simulink model "EV6_LUT_FourWheel_EV6Battery77p4kWh_PowerCorrected"  (R2024a)
settings: Solver=ode4  StartTime=0  StopTime=60  FixedStep=0.001  RelTol=1e-3
PreLoadFcn:
  | VSS_BICYCLE=Simulink.Variant('Dual=0');
  | VSS_DUAL=Simulink.Variant('Dual=1');
  | Dual=1;
  | load('DriveCycle2.mat')
PostLoadFcn:
  | if any(exist('dsrtsu_mdlpostloadfcn', 'file') ~= 0), dsrtsu_mdlpostloadfcn('Execute', bdroot); end
InitFcn:
  | , if any(exist('rtifpga_mdlclblib', 'file') ~= 0), rtifpga_mdlclblib('Init', bdroot); end,
  | , if any(exist('dsmpb_private', 'file') ~= 0), dsmpb_private('dsmpb_mdlclblib', 'Init', bdroot); end,
  | load('DriveCycle2.mat')
model workspace (MAT data in the model file):
  DiffRatio = 10.65
  EV6_2023_BattBranchCapacity_Ah = 55.5236728838
  EV6_2023_BattEnergy_kWh = 77.4
  EV6_2023_BattNominalVoltage_V = 697
  EV6_2023_BattNumCellsParallel = 2
  EV6_2023_BattNumCellsSeries = 192
  EV6_2023_BattOpenVoltCapBpts = [0 0.1 0.2 0.3 0.4 0.5 0.6 0.7 0.8 0.9 1]
  EV6_2023_BattOpenVoltTbl = [2.96762142548 3.40364281191 3.47417488548 3.54470541822 3.61523441014 3.68576186124 3.75628777151 3.82681214095 3.94527005036 4.07101207308 4.2120755254]
  EV6_2023_BattPackCapacity_Ah = 111.047345768
  EV6_2023_BattResistSocBpts = [0 0.2 0.4 0.6 0.8 1]
  EV6_2023_BattResistTbl = [0.0163620057716 0.0118174152018 0.00807187352333 0.00375663957972 0.00266904525531 0.00103635901355 0.0019014404175 0.0172368903217 0.0121226074867 0.00758541551769 0.00474065349228 0.00337561163613 ... (42 elements, 7x6)]
  EV6_2023_BattResistTempBpts = [243.1 253.1 263.1 273.1 283.1 298.1 313.1]
  EV6_2023_InitialPackOCV_V = 726.471714233
  EV6_2023_InitialSOC = 0.638878863672
  EV6_BattCellCapacity_Ah = 60.3
  EV6_BattInitialSOC = 0.638878863672
  EV6_BattOCV_Cell_V = [2.96762142548 3.40364281191 3.47417488548 3.54470541822 3.61523441014 3.68576186124 3.75628777151 3.82681214095 3.94527005036 4.07101207308 4.2120755254]
  EV6_BattOCV_SOC = [0 0.1 0.2 0.3 0.4 0.5 0.6 0.7 0.8 0.9 1]
  EV6_BattPackCapacity_Ah = 120.6
  EV6_BattParallelCells = 2
  EV6_BattResistanceSOC = [0 0.2 0.4 0.6 0.8 1]
  EV6_BattResistanceTable_Ohm = [0.0163620057716 0.0118174152018 0.00807187352333 0.00375663957972 0.00266904525531 0.00103635901355 0.0019014404175 0.0172368903217 0.0121226074867 0.00758541551769 0.00474065349228 0.00337561163613 ... (42 elements, 7x6)]
  EV6_BattResistanceTemp_K = [243.1 253.1 263.1 273.1 283.1 298.1 313.1]
  EV6_BattSeriesCells = 192
  EV6_FinalDriveRatio = 10.65
  EV6_TargetPackResistance_Ohm = 0.132763804608
  Gas = 0.383333333333
undefined symbols (not defined in the file): accel_bp_mps2, AccelCmd, ActTqLF_Nm_, ActTqLR_Nm_, ActTqRF_Nm_, ActTqRR_Nm_, BattChargeLimitMaxPwr, BattChargeLimitSocBpts, BattChargeLimitTbl, BattDischargeLimitSocBpts, BattDischargeLimitTbl, BattDischargeMaxPwr, BrakeMaxPrs, BrakeMaxTrq, ChassisDistCg2FrontAxle, ChassisDistCg2RearAxle, ChassisVehMass, CltchCmd, CoastDown, DecelCmd, DiscIntNeverNeededParam, EnvGravCnst, EnvPrs, EnvTemp, EV6_RegenTorqueGain, EV6_TractionTorqueGain, front_share_regen_3d, front_share_traction_3d, FuelSpecificGrav, GearCmd, h, InitStates, lgSw, limitedMCT, MCT, MtrEffSpdBpts, MtrEffTbl, MtrEffTrqBpts, MtrPwrMax, MtrTrqMax, out_1, pMCT, RealSimPara, Ref_speed, Ref_time, regen_torque_bp_Nm, speed_bp_kph, SteeringCmd, SupvsryCtrlRegenBrkCutOffTbl, SupvsryCtrlRegenSpdBpts, TestScnrioCycleNum, traction_torque_bp_Nm, US06, VEH
libraries: VSIGenLib x65, simulink x54, etargetslib x38, dsmpblib x24, vehdynlibtire x12, autolibshared x11, vehdynlibsuspension x7, vehdynlibtirecommon x7, autolibpowerinfoutils x6, autolibutils x5, autolibsharedcoupling x4, autolibmappedmotor x4
(part 18 of 19)

== system EV6_LUT_FourWheel_EV6Battery77p4kWh_PowerCorrected/Vehicle Under Test1/Vehicle/Vehicle Dynamics/Vehicle 14DOF/Wheels and Tires/VDBS/Veh2Tire/Wheel Angles ==
  steer : Inport
  camber : Inport  Port=2
  Add1 : Sum
  Add2 : Sum
  Constant1 : Constant  Value=pi
  Constant2 : Constant  Value=[pi;0;pi;0].*0+[0;pi;0;pi].*0
  Constant3 : Constant  Value=ones(1,4).*0
  Reshape : Reshape  OutputDimensionality=Row vector (2-D)
  Reshape1 : Reshape  OutputDimensionality=Row vector (2-D)
  Reshape2 : Reshape  OutputDimensionality=Row vector (2-D)
  Vector Concatenate3 : Concatenate  NumInputs=3  Mode=Multidimensional array
  Vehicle : Outport  VectorParamsAs1DForOutWhenUnconnected=off
  wires:
  Add2/1 -> Reshape1/1
  Constant1/1 -> Add2/2
  Add1/1 -> Reshape/1
  steer/1 -> Add1/1
  Reshape2/1 -> Vector Concatenate3/2
  camber/1 -> Add2/1
  Reshape1/1 -> Vector Concatenate3/1
  Reshape/1 -> Vector Concatenate3/3
  Vector Concatenate3/1 -> Vehicle/1
  Constant3/1 -> Reshape2/1
  Constant2/1 -> Add1/2

== system EV6_LUT_FourWheel_EV6Battery77p4kWh_PowerCorrected/Vehicle Under Test1/Vehicle/Vehicle Dynamics/Vehicle 14DOF/Wheels and Tires/VDBS/Veh2Tire/Wheel to Body Transform ==
  VelVeh : Inport  Partition=on  PartitionDimension=2  PartitionWidth=1  PartitionOffset=0
  WheelAngles : Inport  Port=2  Partition=on  PartitionDimension=2  PartitionWidth=1  PartitionOffset=0
  Demux1 : Demux  Outputs=3
  Divide1 : Product  Inputs=**  Multiplication=Matrix(*)
  For Each : ForEach  DisableCoverage=on
  Rotation Angles to Direction Cosine Matrix Retro: ZYX : Subsystem
  Selector : Selector  InputPortWidth=3  IndexOptions=Index vector (dialog)  Indices=[3 2 1]  OutputSizes=1
  xdotWheel : Outport  ConcatenationDimension=1  VectorParamsAs1DForOutWhenUnconnected=off
  ydotWheel : Outport  Port=2  ConcatenationDimension=1  VectorParamsAs1DForOutWhenUnconnected=off
  zdotWheel : Outport  Port=3  ConcatenationDimension=1  VectorParamsAs1DForOutWhenUnconnected=off
  wires:
  Selector/1 -> Rotation Angles to Direction Cosine Matrix Retro: ZYX/1(In1)
  WheelAngles/1 -> Selector/1
  VelVeh/1 -> Divide1/2
  Rotation Angles to Direction Cosine Matrix Retro: ZYX/1(Out1) -> Divide1/1
  Demux1/3 -> zdotWheel/1
  Demux1/2 -> ydotWheel/1
  Demux1/1 -> xdotWheel/1
  Divide1/1 -> Demux1/1

== system EV6_LUT_FourWheel_EV6Battery77p4kWh_PowerCorrected/Vehicle Under Test1/Vehicle/Vehicle Dynamics/Vehicle 7DOF/Longitudinal Wheels 4DOF/Velocity and Vertical Load/Bicycle/Bicycle Fz ==
  In1 : Inport
  Bus Selector6 : BusSelector  OutputSignals=BdyFrm.Forces.Tires.FrntTire.Fz,BdyFrm.Forces.Tires.RearTire.Fz
  Cont LPF : autolibutils/Cont LPF  wc=20*2*pi  AbsoluteTolerance=auto  aMode=2
  Mux5 : Mux
  Saturation : Saturate  UpperLimit=20e3  LowerLimit=1000  ZeroCross=off
  Out1 : Outport  VectorParamsAs1DForOutWhenUnconnected=off
  wires:
  Mux5/1 -> Saturation/1
  Bus Selector6/1 -> Mux5/1, Mux5/2  "<Fz>"
  In1/1 -> Bus Selector6/1
  Bus Selector6/2 -> Mux5/3, Mux5/4  "<Fz>"
  Saturation/1 -> Cont LPF/1
  Cont LPF/1 -> Out1/1

== system EV6_LUT_FourWheel_EV6Battery77p4kWh_PowerCorrected/Vehicle Under Test1/Vehicle/Vehicle Dynamics/Vehicle 7DOF/Longitudinal Wheels 4DOF/Velocity and Vertical Load/Bicycle/Bicycle V ==
  In1 : Inport
  Bus Selector : BusSelector  OutputSignals=BdyFrm.FrntAxl.Vel.xdot,BdyFrm.FrntAxl.Vel.ydot,BdyFrm.FrntAxl.Vel.zdot  OutputAsBus=on
  Bus Selector3 : BusSelector  OutputSignals=BdyFrm.RearAxl.Vel.xdot,BdyFrm.RearAxl.Vel.ydot,BdyFrm.RearAxl.Vel.zdot  OutputAsBus=on
  Bus to Vector1 : BusToVector
  Bus to Vector3 : BusToVector
  Vector Concatenate1 : Concatenate  NumInputs=4  Mode=Multidimensional array  ConcatenateDimension=2
  Out1 : Outport  VectorParamsAs1DForOutWhenUnconnected=off
  wires:
  Vector Concatenate1/1 -> Out1/1
  Bus to Vector3/1 -> Vector Concatenate1/3, Vector Concatenate1/4
  Bus Selector/1 -> Bus to Vector1/1
  In1/1 -> Bus Selector/1, Bus Selector3/1
  Bus to Vector1/1 -> Vector Concatenate1/1, Vector Concatenate1/2
  Bus Selector3/1 -> Bus to Vector3/1

== system EV6_LUT_FourWheel_EV6Battery77p4kWh_PowerCorrected/Vehicle Under Test1/Vehicle/Vehicle Dynamics/Vehicle 7DOF/Longitudinal Wheels 4DOF/Velocity and Vertical Load/Dual/Dual Fz ==
  In1 : Inport
  Bus Selector6 : BusSelector  OutputSignals=BdyFrm.Forces.Tires.FrntTires.Lft.Fz,BdyFrm.Forces.Tires.FrntTires.Rght.Fz,BdyFrm.Forces.Tires.RearTires.Lft.Fz,BdyFrm.Forces.Tires.RearTires.Rght.Fz
  Cont LPF : autolibutils/Cont LPF  wc=20*2*pi  AbsoluteTolerance=auto  aMode=2
  Saturation : Saturate  UpperLimit=20e3  LowerLimit=1000  ZeroCross=off
  Vector Concatenate : Concatenate  NumInputs=4
  Out1 : Outport  VectorParamsAs1DForOutWhenUnconnected=off
  wires:
  Bus Selector6/4 -> Vector Concatenate/4  "<Fz>"
  Bus Selector6/3 -> Vector Concatenate/3  "<Fz>"
  Bus Selector6/1 -> Vector Concatenate/1  "<Fz>"
  Bus Selector6/2 -> Vector Concatenate/2  "<Fz>"
  Vector Concatenate/1 -> Saturation/1
  Cont LPF/1 -> Out1/1
  Saturation/1 -> Cont LPF/1
  In1/1 -> Bus Selector6/1

== system EV6_LUT_FourWheel_EV6Battery77p4kWh_PowerCorrected/Vehicle Under Test1/Vehicle/Vehicle Dynamics/Vehicle 7DOF/Longitudinal Wheels 4DOF/Velocity and Vertical Load/Dual/Dual V ==
  In1 : Inport
  Bus Selector1 : BusSelector  OutputSignals=BdyFrm.FrntAxl.Lft.Vel.xdot,BdyFrm.FrntAxl.Lft.Vel.ydot,BdyFrm.FrntAxl.Lft.Vel.zdot  OutputAsBus=on
  Bus Selector2 : BusSelector  OutputSignals=BdyFrm.FrntAxl.Rght.Vel.xdot,BdyFrm.FrntAxl.Rght.Vel.ydot,BdyFrm.FrntAxl.Rght.Vel.zdot  OutputAsBus=on
  Bus Selector4 : BusSelector  OutputSignals=BdyFrm.RearAxl.Lft.Vel.xdot,BdyFrm.RearAxl.Lft.Vel.ydot,BdyFrm.RearAxl.Lft.Vel.zdot  OutputAsBus=on
  Bus Selector5 : BusSelector  OutputSignals=BdyFrm.RearAxl.Rght.Vel.xdot,BdyFrm.RearAxl.Rght.Vel.ydot,BdyFrm.RearAxl.Rght.Vel.zdot  OutputAsBus=on
  Bus to Vector{5..8} (4 alike) : BusToVector
  Vector Concatenate2 : Concatenate  NumInputs=4  Mode=Multidimensional array  ConcatenateDimension=2
  Out1 : Outport  VectorParamsAs1DForOutWhenUnconnected=off
  wires:
  Vector Concatenate2/1 -> Out1/1
  Bus to Vector7/1 -> Vector Concatenate2/3
  Bus Selector5/1 -> Bus to Vector8/1
  In1/1 -> Bus Selector5/1, Bus Selector4/1, Bus Selector2/1, Bus Selector1/1
  Bus Selector1/1 -> Bus to Vector5/1
  Bus to Vector5/1 -> Vector Concatenate2/1
  Bus Selector4/1 -> Bus to Vector7/1
  Bus to Vector8/1 -> Vector Concatenate2/4
  Bus Selector2/1 -> Bus to Vector6/1
  Bus to Vector6/1 -> Vector Concatenate2/2

== system EV6_LUT_FourWheel_EV6Battery77p4kWh_PowerCorrected/Vehicle Under Test1/Vehicle/Vehicle Dynamics/Vehicle 14DOF/Wheels and Tires/VDBS/Tire2Veh/Wheel to Body Transform/Rotation Angles to Direction Cosine Matrix Retro: ZYX ==
  In1 : Inport
  Fcn : Fcn  Expr=u(5)*u(4)
  Fcn1 : Fcn  Expr=u(5)*u(1)
  Fcn2 : Fcn  Expr=-u(2)
  Fcn3 : Fcn  Expr=u(3)*u(2)*u(4)-u(6)*u(1)
  Fcn4 : Fcn  Expr=u(3)*u(2)*u(1)-u(6)*u(4)
  Fcn5 : Fcn  Expr=u(3)*u(5)
  Fcn6 : Fcn  Expr=u(6)*u(2)*u(4)-u(3)*u(1)
  Fcn7 : Fcn  Expr=u(6)*u(2)*u(1)-u(3)*u(4)
  Fcn8 : Fcn  Expr=u(6)*u(5)
  Mux : Mux  Inputs=2
  SinCos : Trigonometry  Operator=sincos
  Subsystem : Subsystem
  Out1 : Outport
  wires:
  Subsystem/1(Out1) -> Out1/1
  Fcn6/1 -> Subsystem/7(In7)
  Fcn3/1 -> Subsystem/4(In4)
  Fcn2/1 -> Subsystem/3(In3)
  Fcn5/1 -> Subsystem/6(In6)
  In1/1 -> SinCos/1
  Fcn4/1 -> Subsystem/5(In5)
  Fcn/1 -> Subsystem/1(In1)
  Fcn7/1 -> Subsystem/8(In8)
  Fcn8/1 -> Subsystem/9(In9)
  SinCos/1 -> Mux/1
  SinCos/2 -> Mux/2
  Mux/1 -> Fcn4/1, Fcn3/1, Fcn2/1, Fcn1/1, Fcn/1, Fcn5/1, Fcn6/1, Fcn7/1, Fcn8/1
  Fcn1/1 -> Subsystem/2(In2)

== system EV6_LUT_FourWheel_EV6Battery77p4kWh_PowerCorrected/Vehicle Under Test1/Vehicle/Vehicle Dynamics/Vehicle 14DOF/Wheels and Tires/VDBS/Tires/Fiala Tires/Fx ==
  In1 : Inport
  In2 : Inport  Port=2
  In3 : Inport  Port=3
  In4 : Inport  Port=4
  Bus Selector{,1..3} (4 alike) : BusSelector  OutputSignals=Fx
  Vector Concatenate : Concatenate  NumInputs=4
  Out1 : Outport  VectorParamsAs1DForOutWhenUnconnected=off
  wires:
  Vector Concatenate/1 -> Out1/1
  In1/1 -> Bus Selector/1
  Bus Selector/1 -> Vector Concatenate/1  "<Fx>"
  In2/1 -> Bus Selector1/1
  In3/1 -> Bus Selector2/1
  In4/1 -> Bus Selector3/1
  Bus Selector1/1 -> Vector Concatenate/2  "<Fx>"
  Bus Selector2/1 -> Vector Concatenate/3  "<Fx>"
  Bus Selector3/1 -> Vector Concatenate/4  "<Fx>"

== system EV6_LUT_FourWheel_EV6Battery77p4kWh_PowerCorrected/Vehicle Under Test1/Vehicle/Vehicle Dynamics/Vehicle 14DOF/Wheels and Tires/VDBS/Tires/Fiala Tires/Fy ==
  In1 : Inport
  In2 : Inport  Port=2
  In3 : Inport  Port=3
  In4 : Inport  Port=4
  Bus Selector{,1..3} (4 alike) : BusSelector  OutputSignals=Fy
  Vector Concatenate : Concatenate  NumInputs=4
  Out1 : Outport  VectorParamsAs1DForOutWhenUnconnected=off
  wires:
  Bus Selector3/1 -> Vector Concatenate/4  "<Fy>"
  Bus Selector2/1 -> Vector Concatenate/3  "<Fy>"
  Bus Selector1/1 -> Vector Concatenate/2  "<Fy>"
  In4/1 -> Bus Selector3/1
  In3/1 -> Bus Selector2/1
  In2/1 -> Bus Selector1/1
  Bus Selector/1 -> Vector Concatenate/1  "<Fy>"
  In1/1 -> Bus Selector/1
  Vector Concatenate/1 -> Out1/1

== system EV6_LUT_FourWheel_EV6Battery77p4kWh_PowerCorrected/Vehicle Under Test1/Vehicle/Vehicle Dynamics/Vehicle 14DOF/Wheels and Tires/VDBS/Tires/Fiala Tires/Fz ==
  In1 : Inport
  In2 : Inport  Port=2
  In3 : Inport  Port=3
  In4 : Inport  Port=4
  Bus Selector{,1..3} (4 alike) : BusSelector  OutputSignals=Fz
  Vector Concatenate : Concatenate  NumInputs=4
  Out1 : Outport  VectorParamsAs1DForOutWhenUnconnected=off
  wires:
  Bus Selector3/1 -> Vector Concatenate/4  "<Fz>"
  Bus Selector2/1 -> Vector Concatenate/3  "<Fz>"
  Bus Selector1/1 -> Vector Concatenate/2  "<Fz>"
  In4/1 -> Bus Selector3/1
  In3/1 -> Bus Selector2/1
  In2/1 -> Bus Selector1/1
  Bus Selector/1 -> Vector Concatenate/1  "<Fz>"
  In1/1 -> Bus Selector/1
  Vector Concatenate/1 -> Out1/1

== system EV6_LUT_FourWheel_EV6Battery77p4kWh_PowerCorrected/Vehicle Under Test1/Vehicle/Vehicle Dynamics/Vehicle 14DOF/Wheels and Tires/VDBS/Tires/Fiala Tires/Mx ==
  In1 : Inport
  In2 : Inport  Port=2
  In3 : Inport  Port=3
  In4 : Inport  Port=4
  Bus Selector{,1..3} (4 alike) : BusSelector  OutputSignals=Mx
  Vector Concatenate : Concatenate  NumInputs=4
  Out1 : Outport  VectorParamsAs1DForOutWhenUnconnected=off
  wires:
  Bus Selector3/1 -> Vector Concatenate/4  "<Mx>"
  Bus Selector2/1 -> Vector Concatenate/3  "<Mx>"
  Bus Selector1/1 -> Vector Concatenate/2  "<Mx>"
  In4/1 -> Bus Selector3/1
  In3/1 -> Bus Selector2/1
  In2/1 -> Bus Selector1/1
  Bus Selector/1 -> Vector Concatenate/1  "<Mx>"
  In1/1 -> Bus Selector/1
  Vector Concatenate/1 -> Out1/1

== system EV6_LUT_FourWheel_EV6Battery77p4kWh_PowerCorrected/Vehicle Under Test1/Vehicle/Vehicle Dynamics/Vehicle 14DOF/Wheels and Tires/VDBS/Tires/Fiala Tires/My ==
  In1 : Inport
  In2 : Inport  Port=2
  In3 : Inport  Port=3
  In4 : Inport  Port=4
  Bus Selector{,1..3} (4 alike) : BusSelector  OutputSignals=My
  Vector Concatenate : Concatenate  NumInputs=4
  Out1 : Outport  VectorParamsAs1DForOutWhenUnconnected=off
  wires:
  Vector Concatenate/1 -> Out1/1
  In1/1 -> Bus Selector/1
  Bus Selector/1 -> Vector Concatenate/1  "<My>"
  In2/1 -> Bus Selector1/1
  In3/1 -> Bus Selector2/1
  In4/1 -> Bus Selector3/1
  Bus Selector1/1 -> Vector Concatenate/2  "<My>"
  Bus Selector2/1 -> Vector Concatenate/3  "<My>"
  Bus Selector3/1 -> Vector Concatenate/4  "<My>"

== system EV6_LUT_FourWheel_EV6Battery77p4kWh_PowerCorrected/Vehicle Under Test1/Vehicle/Vehicle Dynamics/Vehicle 14DOF/Wheels and Tires/VDBS/Tires/Fiala Tires/Mz ==
  In1 : Inport
  In2 : Inport  Port=2
  In3 : Inport  Port=3
  In4 : Inport  Port=4
  Bus Selector{,1..3} (4 alike) : BusSelector  OutputSignals=Mz
  Vector Concatenate : Concatenate  NumInputs=4
  Out1 : Outport  VectorParamsAs1DForOutWhenUnconnected=off
  wires:
  Vector Concatenate/1 -> Out1/1
  In1/1 -> Bus Selector/1
  Bus Selector/1 -> Vector Concatenate/1  "<Mz>"
  In2/1 -> Bus Selector1/1
  In3/1 -> Bus Selector2/1
  In4/1 -> Bus Selector3/1
  Bus Selector1/1 -> Vector Concatenate/2  "<Mz>"
  Bus Selector2/1 -> Vector Concatenate/3  "<Mz>"
  Bus Selector3/1 -> Vector Concatenate/4  "<Mz>"

== system EV6_LUT_FourWheel_EV6Battery77p4kWh_PowerCorrected/Vehicle Under Test1/Vehicle/Vehicle Dynamics/Vehicle 14DOF/Wheels and Tires/VDBS/Tires/Fiala Tires/Re ==
  In1 : Inport
  In2 : Inport  Port=2
  In3 : Inport  Port=3
  In4 : Inport  Port=4
  Bus Selector{,1..3} (4 alike) : BusSelector  OutputSignals=Re
  Vector Concatenate : Concatenate  NumInputs=4
  Out1 : Outport  VectorParamsAs1DForOutWhenUnconnected=off
  wires:
  Bus Selector3/1 -> Vector Concatenate/4  "<Re>"
  Bus Selector2/1 -> Vector Concatenate/3  "<Re>"
  Bus Selector1/1 -> Vector Concatenate/2  "<Re>"
  In4/1 -> Bus Selector3/1
  In3/1 -> Bus Selector2/1
  In2/1 -> Bus Selector1/1
  Bus Selector/1 -> Vector Concatenate/1  "<Re>"
  In1/1 -> Bus Selector/1
  Vector Concatenate/1 -> Out1/1

== system EV6_LUT_FourWheel_EV6Battery77p4kWh_PowerCorrected/Vehicle Under Test1/Vehicle/Vehicle Dynamics/Vehicle 14DOF/Wheels and Tires/VDBS/Tires/Fiala Tires/alpha ==
  In1 : Inport
  In2 : Inport  Port=2
  In3 : Inport  Port=3
  In4 : Inport  Port=4
  Bus Selector{,1..3} (4 alike) : BusSelector  OutputSignals=Alpha
  Vector Concatenate : Concatenate  NumInputs=4
  Out1 : Outport  VectorParamsAs1DForOutWhenUnconnected=off
  wires:
  Bus Selector3/1 -> Vector Concatenate/4  "<Alpha>"
  Bus Selector2/1 -> Vector Concatenate/3  "<Alpha>"
  Bus Selector1/1 -> Vector Concatenate/2  "<Alpha>"
  In4/1 -> Bus Selector3/1
  In3/1 -> Bus Selector2/1
  In2/1 -> Bus Selector1/1
  Bus Selector/1 -> Vector Concatenate/1  "<Alpha>"
  In1/1 -> Bus Selector/1
  Vector Concatenate/1 -> Out1/1

== system EV6_LUT_FourWheel_EV6Battery77p4kWh_PowerCorrected/Vehicle Under Test1/Vehicle/Vehicle Dynamics/Vehicle 14DOF/Wheels and Tires/VDBS/Tires/Fiala Tires/kappa ==
  In1 : Inport
  In2 : Inport  Port=2
  In3 : Inport  Port=3
  In4 : Inport  Port=4
  Bus Selector{,1..3} (4 alike) : BusSelector  OutputSignals=Kappa
  Vector Concatenate : Concatenate  NumInputs=4
  Out1 : Outport  VectorParamsAs1DForOutWhenUnconnected=off
  wires:
  Vector Concatenate/1 -> Out1/1
  In1/1 -> Bus Selector/1
  Bus Selector/1 -> Vector Concatenate/1  "<Kappa>"
  In2/1 -> Bus Selector1/1
  In3/1 -> Bus Selector2/1
  In4/1 -> Bus Selector3/1
  Bus Selector1/1 -> Vector Concatenate/2  "<Kappa>"
  Bus Selector2/1 -> Vector Concatenate/3  "<Kappa>"
  Bus Selector3/1 -> Vector Concatenate/4  "<Kappa>"

== system EV6_LUT_FourWheel_EV6Battery77p4kWh_PowerCorrected/Vehicle Under Test1/Vehicle/Vehicle Dynamics/Vehicle 14DOF/Wheels and Tires/VDBS/Tires/Fiala Tires/omega ==
  In1 : Inport
  In2 : Inport  Port=2
  In3 : Inport  Port=3
  In4 : Inport  Port=4
  Bus Selector{,1..3} (4 alike) : BusSelector  OutputSignals=Omega
  Vector Concatenate : Concatenate  NumInputs=4
  Out1 : Outport  VectorParamsAs1DForOutWhenUnconnected=off
  wires:
  Vector Concatenate/1 -> Out1/1
  Bus Selector3/1 -> Vector Concatenate/4  "<Omega>"
  Bus Selector2/1 -> Vector Concatenate/3  "<Omega>"
  Bus Selector1/1 -> Vector Concatenate/2  "<Omega>"
  In4/1 -> Bus Selector3/1
  In3/1 -> Bus Selector2/1
  In2/1 -> Bus Selector1/1
  Bus Selector/1 -> Vector Concatenate/1  "<Omega>"
  In1/1 -> Bus Selector/1

== system EV6_LUT_FourWheel_EV6Battery77p4kWh_PowerCorrected/Vehicle Under Test1/Vehicle/Vehicle Dynamics/Vehicle 14DOF/Wheels and Tires/VDBS/Tires/Fiala Tires/z ==
  In1 : Inport
  In2 : Inport  Port=2
  In3 : Inport  Port=3
  In4 : Inport  Port=4
  Bus Selector{,1..3} (4 alike) : BusSelector  OutputSignals=z
  Vector Concatenate : Concatenate  NumInputs=4
  Out1 : Outport  VectorParamsAs1DForOutWhenUnconnected=off
  wires:
  Vector Concatenate/1 -> Out1/1
  In1/1 -> Bus Selector/1
  Bus Selector/1 -> Vector Concatenate/1  "<z>"
  In2/1 -> Bus Selector1/1
  In3/1 -> Bus Selector2/1
  In4/1 -> Bus Selector3/1
  Bus Selector1/1 -> Vector Concatenate/2  "<z>"
  Bus Selector2/1 -> Vector Concatenate/3  "<z>"
  Bus Selector3/1 -> Vector Concatenate/4  "<z>"

== system EV6_LUT_FourWheel_EV6Battery77p4kWh_PowerCorrected/Vehicle Under Test1/Vehicle/Vehicle Dynamics/Vehicle 14DOF/Wheels and Tires/VDBS/Tires/Fiala Tires/zdot ==
  In1 : Inport
  In2 : Inport  Port=2
  In3 : Inport  Port=3
  In4 : Inport  Port=4
  Bus Selector{,1..3} (4 alike) : BusSelector  OutputSignals=zdot
  Vector Concatenate : Concatenate  NumInputs=4
  Out1 : Outport  VectorParamsAs1DForOutWhenUnconnected=off
  wires:
  Bus Selector3/1 -> Vector Concatenate/4  "<zdot>"
  Bus Selector2/1 -> Vector Concatenate/3  "<zdot>"
  Bus Selector1/1 -> Vector Concatenate/2  "<zdot>"
  In4/1 -> Bus Selector3/1
  In3/1 -> Bus Selector2/1
  In2/1 -> Bus Selector1/1
  Bus Selector/1 -> Vector Concatenate/1  "<zdot>"
  In1/1 -> Bus Selector/1
  Vector Concatenate/1 -> Out1/1

== system EV6_LUT_FourWheel_EV6Battery77p4kWh_PowerCorrected/Vehicle Under Test1/Vehicle/Vehicle Dynamics/Vehicle 14DOF/Wheels and Tires/VDBS/Tires/MF Tires/Fx ==
  In1 : Inport
  In2 : Inport  Port=2
  In3 : Inport  Port=3
  In4 : Inport  Port=4
  Bus Selector{,1..3} (4 alike) : BusSelector  OutputSignals=Fx
  Vector Concatenate : Concatenate  NumInputs=4
  Out1 : Outport  VectorParamsAs1DForOutWhenUnconnected=off
  wires:
  Vector Concatenate/1 -> Out1/1
  In1/1 -> Bus Selector/1
  Bus Selector/1 -> Vector Concatenate/1  "<Fx>"
  In2/1 -> Bus Selector1/1
  In3/1 -> Bus Selector2/1
  In4/1 -> Bus Selector3/1
  Bus Selector1/1 -> Vector Concatenate/2  "<Fx>"
  Bus Selector2/1 -> Vector Concatenate/3  "<Fx>"
  Bus Selector3/1 -> Vector Concatenate/4  "<Fx>"

== system EV6_LUT_FourWheel_EV6Battery77p4kWh_PowerCorrected/Vehicle Under Test1/Vehicle/Vehicle Dynamics/Vehicle 14DOF/Wheels and Tires/VDBS/Tires/MF Tires/Fy ==
  In1 : Inport
  In2 : Inport  Port=2
  In3 : Inport  Port=3
  In4 : Inport  Port=4
  Bus Selector{,1..3} (4 alike) : BusSelector  OutputSignals=Fy
  Vector Concatenate : Concatenate  NumInputs=4
  Out1 : Outport  VectorParamsAs1DForOutWhenUnconnected=off
  wires:
  Bus Selector3/1 -> Vector Concatenate/4  "<Fy>"
  Bus Selector2/1 -> Vector Concatenate/3  "<Fy>"
  Bus Selector1/1 -> Vector Concatenate/2  "<Fy>"
  In4/1 -> Bus Selector3/1
  In3/1 -> Bus Selector2/1
  In2/1 -> Bus Selector1/1
  Bus Selector/1 -> Vector Concatenate/1  "<Fy>"
  In1/1 -> Bus Selector/1
  Vector Concatenate/1 -> Out1/1

== system EV6_LUT_FourWheel_EV6Battery77p4kWh_PowerCorrected/Vehicle Under Test1/Vehicle/Vehicle Dynamics/Vehicle 14DOF/Wheels and Tires/VDBS/Tires/MF Tires/Fz ==
  In1 : Inport
  In2 : Inport  Port=2
  In3 : Inport  Port=3
  In4 : Inport  Port=4
  Bus Selector{,1..3} (4 alike) : BusSelector  OutputSignals=Fz
  Vector Concatenate : Concatenate  NumInputs=4
  Out1 : Outport  VectorParamsAs1DForOutWhenUnconnected=off
  wires:
  Bus Selector3/1 -> Vector Concatenate/4  "<Fz>"
  Bus Selector2/1 -> Vector Concatenate/3  "<Fz>"
  Bus Selector1/1 -> Vector Concatenate/2  "<Fz>"
  In4/1 -> Bus Selector3/1
  In3/1 -> Bus Selector2/1
  In2/1 -> Bus Selector1/1
  Bus Selector/1 -> Vector Concatenate/1  "<Fz>"
  In1/1 -> Bus Selector/1
  Vector Concatenate/1 -> Out1/1

== system EV6_LUT_FourWheel_EV6Battery77p4kWh_PowerCorrected/Vehicle Under Test1/Vehicle/Vehicle Dynamics/Vehicle 14DOF/Wheels and Tires/VDBS/Tires/MF Tires/Mx ==
  In1 : Inport
  In2 : Inport  Port=2
  In3 : Inport  Port=3
  In4 : Inport  Port=4
  Bus Selector{,1..3} (4 alike) : BusSelector  Commented=on  OutputSignals=Mx
  Vector Concatenate : Concatenate  NumInputs=4
  Out1 : Outport  VectorParamsAs1DForOutWhenUnconnected=off
  wires:
  In4/1 -> Vector Concatenate/4
  In3/1 -> Vector Concatenate/3
  In2/1 -> Vector Concatenate/2
  In1/1 -> Vector Concatenate/1
  Bus Selector1/1 -> ?  "<Mx>"
  ? -> Bus Selector3/1
  ? -> Bus Selector/1
  Bus Selector2/1 -> ?  "<Mx>"
  Bus Selector/1 -> ?  "<Mx>"
  Bus Selector3/1 -> ?  "<Mx>"
  ? -> Bus Selector1/1
  ? -> Bus Selector2/1
  Vector Concatenate/1 -> Out1/1

== system EV6_LUT_FourWheel_EV6Battery77p4kWh_PowerCorrected/Vehicle Under Test1/Vehicle/Vehicle Dynamics/Vehicle 14DOF/Wheels and Tires/VDBS/Tires/MF Tires/My ==
  In1 : Inport
  In2 : Inport  Port=2
  In3 : Inport  Port=3
  In4 : Inport  Port=4
  Bus Selector{,1..3} (4 alike) : BusSelector  OutputSignals=My
  Vector Concatenate : Concatenate  NumInputs=4
  Out1 : Outport  VectorParamsAs1DForOutWhenUnconnected=off
  wires:
  Vector Concatenate/1 -> Out1/1
  In1/1 -> Bus Selector/1
  Bus Selector/1 -> Vector Concatenate/1  "<My>"
  In2/1 -> Bus Selector1/1
  In3/1 -> Bus Selector2/1
  In4/1 -> Bus Selector3/1
  Bus Selector1/1 -> Vector Concatenate/2  "<My>"
  Bus Selector2/1 -> Vector Concatenate/3  "<My>"
  Bus Selector3/1 -> Vector Concatenate/4  "<My>"

== system EV6_LUT_FourWheel_EV6Battery77p4kWh_PowerCorrected/Vehicle Under Test1/Vehicle/Vehicle Dynamics/Vehicle 14DOF/Wheels and Tires/VDBS/Tires/MF Tires/Mz ==
  In1 : Inport
  In2 : Inport  Port=2
  In3 : Inport  Port=3
  In4 : Inport  Port=4
  Bus Selector{,1..3} (4 alike) : BusSelector  Commented=on  OutputSignals=Mz
  Vector Concatenate : Concatenate  NumInputs=4
  Out1 : Outport  VectorParamsAs1DForOutWhenUnconnected=off
  wires:
  In4/1 -> Vector Concatenate/4
  In3/1 -> Vector Concatenate/3
  In2/1 -> Vector Concatenate/2
  In1/1 -> Vector Concatenate/1
  Bus Selector1/1 -> ?  "<Mz>"
  Bus Selector/1 -> ?  "<Mz>"
  ? -> Bus Selector3/1
  Bus Selector3/1 -> ?  "<Mz>"
  ? -> Bus Selector2/1
  ? -> Bus Selector1/1
  Bus Selector2/1 -> ?  "<Mz>"
  ? -> Bus Selector/1
  Vector Concatenate/1 -> Out1/1

== system EV6_LUT_FourWheel_EV6Battery77p4kWh_PowerCorrected/Vehicle Under Test1/Vehicle/Vehicle Dynamics/Vehicle 14DOF/Wheels and Tires/VDBS/Tires/MF Tires/Re ==
  In1 : Inport
  In2 : Inport  Port=2
  In3 : Inport  Port=3
  In4 : Inport  Port=4
  Bus Selector{,1..3} (4 alike) : BusSelector  OutputSignals=Re
  Vector Concatenate : Concatenate  NumInputs=4
  Out1 : Outport  VectorParamsAs1DForOutWhenUnconnected=off
  wires:
  Bus Selector3/1 -> Vector Concatenate/4  "<Re>"
  Bus Selector2/1 -> Vector Concatenate/3  "<Re>"
  Bus Selector1/1 -> Vector Concatenate/2  "<Re>"
  In4/1 -> Bus Selector3/1
  In3/1 -> Bus Selector2/1
  In2/1 -> Bus Selector1/1
  Bus Selector/1 -> Vector Concatenate/1  "<Re>"
  In1/1 -> Bus Selector/1
  Vector Concatenate/1 -> Out1/1

== system EV6_LUT_FourWheel_EV6Battery77p4kWh_PowerCorrected/Vehicle Under Test1/Vehicle/Vehicle Dynamics/Vehicle 14DOF/Wheels and Tires/VDBS/Tires/MF Tires/alpha ==
  In1 : Inport
  In2 : Inport  Port=2
  In3 : Inport  Port=3
  In4 : Inport  Port=4
  Bus Selector{,1..3} (4 alike) : BusSelector  OutputSignals=Alpha
  Vector Concatenate : Concatenate  NumInputs=4
  Out1 : Outport  VectorParamsAs1DForOutWhenUnconnected=off
  wires:
  Bus Selector3/1 -> Vector Concatenate/4  "<Alpha>"
  Bus Selector2/1 -> Vector Concatenate/3  "<Alpha>"
  Bus Selector1/1 -> Vector Concatenate/2  "<Alpha>"
  In4/1 -> Bus Selector3/1
  In3/1 -> Bus Selector2/1
  In2/1 -> Bus Selector1/1
  Bus Selector/1 -> Vector Concatenate/1  "<Alpha>"
  In1/1 -> Bus Selector/1
  Vector Concatenate/1 -> Out1/1

== system EV6_LUT_FourWheel_EV6Battery77p4kWh_PowerCorrected/Vehicle Under Test1/Vehicle/Vehicle Dynamics/Vehicle 14DOF/Wheels and Tires/VDBS/Tires/MF Tires/kappa ==
  In1 : Inport
  In2 : Inport  Port=2
  In3 : Inport  Port=3
  In4 : Inport  Port=4
  Bus Selector{,1..3} (4 alike) : BusSelector  OutputSignals=Kappa
  Vector Concatenate : Concatenate  NumInputs=4
  Out1 : Outport  VectorParamsAs1DForOutWhenUnconnected=off
  wires:
  Vector Concatenate/1 -> Out1/1
  In1/1 -> Bus Selector/1
  Bus Selector/1 -> Vector Concatenate/1  "<Kappa>"
  In2/1 -> Bus Selector1/1
  In3/1 -> Bus Selector2/1
  In4/1 -> Bus Selector3/1
  Bus Selector1/1 -> Vector Concatenate/2  "<Kappa>"
  Bus Selector2/1 -> Vector Concatenate/3  "<Kappa>"
  Bus Selector3/1 -> Vector Concatenate/4  "<Kappa>"

== system EV6_LUT_FourWheel_EV6Battery77p4kWh_PowerCorrected/Vehicle Under Test1/Vehicle/Vehicle Dynamics/Vehicle 14DOF/Wheels and Tires/VDBS/Tires/MF Tires/omega ==
  In1 : Inport
  In2 : Inport  Port=2
  In3 : Inport  Port=3
  In4 : Inport  Port=4
  Abs{,1..3} (4 alike) : Abs  SaturateOnIntegerOverflow=off
  Bus Selector{,1..3} (4 alike) : BusSelector  OutputSignals=Omega
  Constant : Constant  Value=0
  Rate Limiter{4..7} (4 alike) : RateLimiter  Commented=on  RisingSlewLimit=3  FallingSlewLimit=-3  SampleTimeMode=inherited
  Scope : Scope  NumInputPorts=2
  Scope1 : Scope  NumInputPorts=4
  Switch{1..4} (4 alike) : Switch  Criteria=u2 > Threshold  Threshold=0.11  SaturateOnIntegerOverflow=off  InputSameDT=off
  Transfer Fcn{,1..3} (4 alike) : TransferFcn  Denominator=[0.1 1]
  Vector Concatenate : Concatenate  NumInputs=4
  Out1 : Outport  VectorParamsAs1DForOutWhenUnconnected=off
  wires:
  Transfer Fcn/1 -> Abs/1, Switch1/1
  Bus Selector1/1 -> Transfer Fcn1/1, Scope1/2  "<Omega>"
  Transfer Fcn2/1 -> Switch3/1, Abs2/1
  Abs1/1 -> Switch2/2
  Abs/1 -> Switch1/2
  Switch1/1 -> Scope/2, Vector Concatenate/1
  Abs3/1 -> Switch4/2
  Constant/1 -> Switch1/3, Switch2/3, Switch3/3, Switch4/3
  Transfer Fcn1/1 -> Switch2/1, Abs1/1
  Transfer Fcn3/1 -> Switch4/1, Abs3/1
  Switch2/1 -> Vector Concatenate/2
  Switch4/1 -> Vector Concatenate/4
  Bus Selector/1 -> Scope/1, Scope1/1, Transfer Fcn/1  "<Omega>"
  Bus Selector2/1 -> Scope1/3, Transfer Fcn2/1  "<Omega>"
  Bus Selector3/1 -> Scope1/4, Transfer Fcn3/1  "<Omega>"
  Switch3/1 -> Vector Concatenate/3
  Abs2/1 -> Switch3/2
  Vector Concatenate/1 -> Out1/1
  In4/1 -> Bus Selector3/1
  In3/1 -> Bus Selector2/1
  In2/1 -> Bus Selector1/1
  In1/1 -> Bus Selector/1

== system EV6_LUT_FourWheel_EV6Battery77p4kWh_PowerCorrected/Vehicle Under Test1/Vehicle/Vehicle Dynamics/Vehicle 14DOF/Wheels and Tires/VDBS/Tires/MF Tires/omega1 ==
  In1 : Inport
  In2 : Inport  Port=2
  In3 : Inport  Port=3
  In4 : Inport  Port=4
  Abs{,1..3} (4 alike) : Abs  SaturateOnIntegerOverflow=off
  Constant : Constant  Value=0
  Rate Limiter{,1..3} (4 alike) : RateLimiter  RisingSlewLimit=5  FallingSlewLimit=-5  SampleTimeMode=inherited
  Switch{1..4} (4 alike) : Switch  Criteria=u2 > Threshold  Threshold=0.11  SaturateOnIntegerOverflow=off  InputSameDT=off
  Transfer Fcn{,1..3} (4 alike) : TransferFcn  Denominator=[0.1 1]
  Vector Concatenate : Concatenate  NumInputs=4
  Out1 : Outport  VectorParamsAs1DForOutWhenUnconnected=off
  wires:
  Transfer Fcn/1 -> Abs/1, Switch1/1
  In2/1 -> Rate Limiter1/1
  Rate Limiter3/1 -> Transfer Fcn3/1
  Transfer Fcn2/1 -> Switch3/1, Abs2/1
  Abs1/1 -> Switch2/2
  Abs/1 -> Switch1/2
  Switch1/1 -> Vector Concatenate/1
  Abs3/1 -> Switch4/2
  Constant/1 -> Switch1/3, Switch2/3, Switch3/3, Switch4/3
  Transfer Fcn1/1 -> Switch2/1, Abs1/1
  Transfer Fcn3/1 -> Switch4/1, Abs3/1
  Rate Limiter/1 -> Transfer Fcn/1
  Switch2/1 -> Vector Concatenate/2
  Switch4/1 -> Vector Concatenate/4
  In1/1 -> Rate Limiter/1
  In3/1 -> Rate Limiter2/1
  Rate Limiter2/1 -> Transfer Fcn2/1
  Rate Limiter1/1 -> Transfer Fcn1/1
  In4/1 -> Rate Limiter3/1
  Switch3/1 -> Vector Concatenate/3
  Abs2/1 -> Switch3/2
  Vector Concatenate/1 -> Out1/1

== system EV6_LUT_FourWheel_EV6Battery77p4kWh_PowerCorrected/Vehicle Under Test1/Vehicle/Vehicle Dynamics/Vehicle 14DOF/Wheels and Tires/VDBS/Tires/MF Tires/z ==
  In1 : Inport
  In2 : Inport  Port=2
  In3 : Inport  Port=3
  In4 : Inport  Port=4
  Bus Selector{,1..3} (4 alike) : BusSelector  OutputSignals=z
  Vector Concatenate : Concatenate  NumInputs=4
  Out1 : Outport  VectorParamsAs1DForOutWhenUnconnected=off
  wires:
  Vector Concatenate/1 -> Out1/1
  In1/1 -> Bus Selector/1
  Bus Selector/1 -> Vector Concatenate/1  "<z>"
  In2/1 -> Bus Selector1/1
  In3/1 -> Bus Selector2/1
  In4/1 -> Bus Selector3/1
  Bus Selector1/1 -> Vector Concatenate/2  "<z>"
  Bus Selector2/1 -> Vector Concatenate/3  "<z>"
  Bus Selector3/1 -> Vector Concatenate/4  "<z>"

== system EV6_LUT_FourWheel_EV6Battery77p4kWh_PowerCorrected/Vehicle Under Test1/Vehicle/Vehicle Dynamics/Vehicle 14DOF/Wheels and Tires/VDBS/Tires/MF Tires/zdot ==
  In1 : Inport
  In2 : Inport  Port=2
  In3 : Inport  Port=3
  In4 : Inport  Port=4
  Bus Selector{,1..3} (4 alike) : BusSelector  OutputSignals=zdot
  Vector Concatenate : Concatenate  NumInputs=4
  Out1 : Outport  VectorParamsAs1DForOutWhenUnconnected=off
  wires:
  Bus Selector3/1 -> Vector Concatenate/4  "<zdot>"
  Bus Selector2/1 -> Vector Concatenate/3  "<zdot>"
  Bus Selector1/1 -> Vector Concatenate/2  "<zdot>"
  In4/1 -> Bus Selector3/1
  In3/1 -> Bus Selector2/1
  In2/1 -> Bus Selector1/1
  Bus Selector/1 -> Vector Concatenate/1  "<zdot>"
  In1/1 -> Bus Selector/1
  Vector Concatenate/1 -> Out1/1

== system EV6_LUT_FourWheel_EV6Battery77p4kWh_PowerCorrected/Vehicle Under Test1/Vehicle/Vehicle Dynamics/Vehicle 14DOF/Wheels and Tires/VDBS/Veh2Tire/Wheel to Body Transform/Rotation Angles to Direction Cosine Matrix Retro: ZYX ==
  In1 : Inport
  Fcn : Fcn  Expr=u(5)*u(4)
  Fcn1 : Fcn  Expr=u(5)*u(1)
  Fcn2 : Fcn  Expr=-u(2)
  Fcn3 : Fcn  Expr=u(3)*u(2)*u(4)-u(6)*u(1)
  Fcn4 : Fcn  Expr=u(3)*u(2)*u(1)-u(6)*u(4)
  Fcn5 : Fcn  Expr=u(3)*u(5)
  Fcn6 : Fcn  Expr=u(6)*u(2)*u(4)-u(3)*u(1)
  Fcn7 : Fcn  Expr=u(6)*u(2)*u(1)-u(3)*u(4)
  Fcn8 : Fcn  Expr=u(6)*u(5)
  Mux : Mux  Inputs=2
  SinCos : Trigonometry  Operator=sincos
  Subsystem : Subsystem
  Out1 : Outport
  wires:
  Subsystem/1(Out1) -> Out1/1
  Fcn6/1 -> Subsystem/7(In7)
  Fcn3/1 -> Subsystem/4(In4)
  Fcn2/1 -> Subsystem/3(In3)
  Fcn5/1 -> Subsystem/6(In6)
  In1/1 -> SinCos/1
  Fcn4/1 -> Subsystem/5(In5)
  Fcn/1 -> Subsystem/1(In1)
  Fcn7/1 -> Subsystem/8(In8)
  Fcn8/1 -> Subsystem/9(In9)
  SinCos/1 -> Mux/1
  SinCos/2 -> Mux/2
  Mux/1 -> Fcn4/1, Fcn3/1, Fcn2/1, Fcn1/1, Fcn/1, Fcn5/1, Fcn6/1, Fcn7/1, Fcn8/1
  Fcn1/1 -> Subsystem/2(In2)

== system EV6_LUT_FourWheel_EV6Battery77p4kWh_PowerCorrected/Vehicle Under Test1/Vehicle/Vehicle Dynamics/Vehicle 14DOF/Wheels and Tires/VDBS/Tire2Veh/Wheel to Body Transform/Rotation Angles to Direction Cosine Matrix Retro: ZYX/Subsystem ==
  In1 : Inport
  In2 : Inport  Port=2
  In3 : Inport  Port=3
  In4 : Inport  Port=4
  In5 : Inport  Port=5
  In6 : Inport  Port=6
  In7 : Inport  Port=7
  In8 : Inport  Port=8
  In9 : Inport  Port=9
  Reshape : Reshape  OutputDimensionality=Customize  OutputDimensions=[3, 3]
  Vector Concatenate : Concatenate  NumInputs=9
  Out1 : Outport
  wires:
  In9/1 -> Vector Concatenate/9
  In6/1 -> Vector Concatenate/8
  In3/1 -> Vector Concatenate/7
  In8/1 -> Vector Concatenate/6
  In5/1 -> Vector Concatenate/5
  In2/1 -> Vector Concatenate/4
  In7/1 -> Vector Concatenate/3
  In4/1 -> Vector Concatenate/2
  In1/1 -> Vector Concatenate/1
  Vector Concatenate/1 -> Reshape/1
  Reshape/1 -> Out1/1

== system EV6_LUT_FourWheel_EV6Battery77p4kWh_PowerCorrected/Vehicle Under Test1/Vehicle/Vehicle Dynamics/Vehicle 14DOF/Wheels and Tires/VDBS/Veh2Tire/Wheel to Body Transform/Rotation Angles to Direction Cosine Matrix Retro: ZYX/Subsystem ==
  In1 : Inport
  In2 : Inport  Port=2
  In3 : Inport  Port=3
  In4 : Inport  Port=4
  In5 : Inport  Port=5
  In6 : Inport  Port=6
  In7 : Inport  Port=7
  In8 : Inport  Port=8
  In9 : Inport  Port=9
  Reshape : Reshape  OutputDimensionality=Customize  OutputDimensions=[3, 3]
  Vector Concatenate : Concatenate  NumInputs=9
  Out1 : Outport
  wires:
  In9/1 -> Vector Concatenate/9
  In6/1 -> Vector Concatenate/8
  In3/1 -> Vector Concatenate/7
  In8/1 -> Vector Concatenate/6
  In5/1 -> Vector Concatenate/5
  In2/1 -> Vector Concatenate/4
  In7/1 -> Vector Concatenate/3
  In4/1 -> Vector Concatenate/2
  In1/1 -> Vector Concatenate/1
  Vector Concatenate/1 -> Reshape/1
  Reshape/1 -> Out1/1

== matlab function EV6_LUT_FourWheel_EV6Battery77p4kWh_PowerCorrected/RealSim1/MATLAB Function3 ==
  data: simState input; connectionState input; timeSimulator input; timeStepSimulator output; timeStepSimulatorPrevious input; timeStepTrigger output
function [timeStepSimulator, timeStepTrigger]  = fcn(simState, connectionState, timeSimulator, timeStepSimulatorPrevious)


if simState && abs(connectionState-3) < 1e-5 && (timeSimulator >= timeStepSimulatorPrevious + 0.1 - 1e-5 || abs(timeSimulator) < 1e-5)
    timeStepSimulator = timeSimulator;
    timeStepTrigger = 1;
else
    timeStepSimulator = timeStepSimulatorPrevious;
    timeStepTrigger = 0;
end

== matlab function EV6_LUT_FourWheel_EV6Battery77p4kWh_PowerCorrected/RealSim1/MATLAB Function ==
  data: strUint8Vec input; intVal output double; strLen input
function intVal = strVec2Int(strUint8Vec, strLen)

    strVec = blanks(50);
    for i = 1:strLen
       strVec(i) = strUint8Vec(i); 
    end
    if strLen > 0
        intVal = real(str2double(strVec(1:strLen)));
    else
        intVal = -1;
    end

== matlab function EV6_LUT_FourWheel_EV6Battery77p4kWh_PowerCorrected/RealSim1/MATLAB Function1 ==
  data: strUint8Vec input; intVal output double; strLen input
function intVal = strVec2Int(strUint8Vec, strLen)

    strVec = blanks(50);
    for i = 1:strLen
       strVec(i) = strUint8Vec(i); 
    end
    if strLen > 0
        intVal = real(str2double(strVec(1:strLen)));
    else
        intVal = -1;
    end

== matlab function EV6_LUT_FourWheel_EV6Battery77p4kWh_PowerCorrected/RealSim1/MATLAB Function2 ==
  data: signalLightId input uint8 size=[1 50]; signalLightIdString output string; signalLightIdLength input
function signalLightIdString = fcn(signalLightId, signalLightIdLength)

signalLightIdString = string(char(signalLightId));

== matlab function EV6_LUT_FourWheel_EV6Battery77p4kWh_PowerCorrected/RealSim1/MATLAB Function4 ==
  data: simState input; simulatorStartTime output; simStatePrevious input; connectionState input; simulationTime input; simState output
function [simulatorStartTime, simState] = fcn(simState, simStatePrevious, connectionState, simulationTime)


if abs(simState - 1) < 1e-5 && abs(simStatePrevious) < 1e-5 && abs(connectionState-3) < 1e-5
    % set connectionState and start time
    simulatorStartTime = simulationTime;
else
    simulatorStartTime = 0;
end

== matlab function EV6_LUT_FourWheel_EV6Battery77p4kWh_PowerCorrected/RealSim2/MATLAB Function ==
  data: strUint8Vec input; intVal output double; strLen input
function intVal = strVec2Int(strUint8Vec, strLen)

    strVec = blanks(50);
    for i = 1:strLen
       strVec(i) = strUint8Vec(i); 
    end
    if strLen > 0
        intVal = real(str2double(strVec(1:strLen)));
    else
        intVal = -1;
    end

== matlab function EV6_LUT_FourWheel_EV6Battery77p4kWh_PowerCorrected/RealSim2/MATLAB Function1 ==
  data: strUint8Vec input; intVal output double; strLen input
function intVal = strVec2Int(strUint8Vec, strLen)

    strVec = blanks(50);
    for i = 1:strLen
       strVec(i) = strUint8Vec(i); 
    end
    if strLen > 0
        intVal = real(str2double(strVec(1:strLen)));
    else
        intVal = -1;
    end

== matlab function EV6_LUT_FourWheel_EV6Battery77p4kWh_PowerCorrected/RealSim2/MATLAB Function2 ==
  data: signalLightId input uint8 size=[1 50]; signalLightIdString output string; signalLightIdLength input
function signalLightIdString = fcn(signalLightId, signalLightIdLength)

signalLightIdString = string(char(signalLightId));

== matlab function EV6_LUT_FourWheel_EV6Battery77p4kWh_PowerCorrected/RealSim2/MATLAB Function3 ==
  data: simState input; connectionState input; timeSimulator input; timeStepSimulator output; timeStepSimulatorPrevious input; timeStepTrigger output
function [timeStepSimulator, timeStepTrigger]  = fcn(simState, connectionState, timeSimulator, timeStepSimulatorPrevious)


if simState && abs(connectionState-3) < 1e-5 && (timeSimulator >= timeStepSimulatorPrevious + 0.1 - 1e-5 || abs(timeSimulator) < 1e-5)
    timeStepSimulator = timeSimulator;
    timeStepTrigger = 1;
else
    timeStepSimulator = timeStepSimulatorPrevious;
    timeStepTrigger = 0;
end

== matlab function EV6_LUT_FourWheel_EV6Battery77p4kWh_PowerCorrected/RealSim2/MATLAB Function4 ==
  data: simState input; simulatorStartTime output; simStatePrevious input; connectionState input; simulationTime input; simState output
function [simulatorStartTime, simState] = fcn(simState, simStatePrevious, connectionState, simulationTime)


if abs(simState - 1) < 1e-5 && abs(simStatePrevious) < 1e-5 && abs(connectionState-3) < 1e-5
    % set connectionState and start time
    simulatorStartTime = simulationTime;
else
    simulatorStartTime = 0;
end

== stateflow chart EV6_LUT_FourWheel_EV6Battery77p4kWh_PowerCorrected/Vehicle Under Test1/Vehicle/Actuation and Outputs/MOOG Brake Actuator/MOOG Interface/MOOG State Machine ==
  state MainStateMachine [parallel]
    settings: executionOrder=2
    state Learning
      state LearnMinStop
        en:
        state BackStopCmd
          en:
          MoogOpMode=21 ;
          PositionCmd=-100000;
        state BackStopReached
          en:
          MoogOpMode=22;
          PositionCmd=0;
        state BackStopSettle
          en:
          MoogOpMode=23;
          MinStop=ActualPosition_cnt;
          PositionCmd=0;
        (default) -> MainStateMachine.Learning.LearnMinStop.BackStopCmd
        MainStateMachine.Learning.LearnMinStop.BackStopCmd -> MainStateMachine.Learning.LearnMinStop.BackStopReached : [bitand(StatusWord,8)]
        MainStateMachine.Learning.LearnMinStop.BackStopReached -> MainStateMachine.Learning.LearnMinStop.BackStopSettle : after(2,sec)
      state StartLearning
        en:
        MoogOpMode=11;
        PositionCmd=0;
        MinStop=-200000;
        MaxStop=200000;
      state LearnMaxStop
        en:
        state BackStopCmd
          en:
          MoogOpMode=31;
          PositionCmd=100000;
        state BackStopReached
          en:
          MoogOpMode=32;
          PositionCmd=0;
        state BackStopSettle
          en:
          MoogOpMode=33;
          MaxStop=ActualPosition_cnt;
          PositionCmd=0;
        (default) -> MainStateMachine.Learning.LearnMaxStop.BackStopCmd
        MainStateMachine.Learning.LearnMaxStop.BackStopCmd -> MainStateMachine.Learning.LearnMaxStop.BackStopReached : [bitand(StatusWord,8)]
        MainStateMachine.Learning.LearnMaxStop.BackStopReached -> MainStateMachine.Learning.LearnMaxStop.BackStopSettle : after(2,sec)
      state EndLearning
        en:
        MoogOpMode=41;
        PositionCmd=0;
        LearningComplete=1;
        FaultCntr=0;
      (default) -> StartLearning
      StartLearning -> LearnMinStop : after(0.5,sec)[InitComplete ==1]
      LearnMinStop -> LearnMaxStop : after(1,sec)[InitComplete ==1  && MinStop ~=-200000]
      LearnMaxStop -> EndLearning : after(1,sec)[InitComplete ==1  && MaxStop ~=200000 && ((MaxStop-MinStop)>ActuatorMinTravelForReady)]
    state NormalOperation
      state LearningNotComplete
        en:
        MoogOpMode=101;
        Actuator_Ready=0;
        du:
        PositionCmd=0;
      state LearningComplete
        en:
        MoogOpMode=102;
        Actuator_Ready=1;
        du:
        PositionCmd=TargetPosition_cnt;
      (default) -> LearningNotComplete
      LearningNotComplete -> LearningComplete : after(1,sec)[LearningComplete==1]
    MainStateMachine.Learning.LearnMaxStop.BackStopSettle -> NormalOperation : after(10,sec)
    Learning -> NormalOperation : after(1,sec)[LearningComplete==1]
    NormalOperation -> Learning : [PositionLearningTrigger==1]{Actuator_Ready =0;
        | LearningComplete=0}
    (default) -> NormalOperation : {Actuator_Ready =0;
        | LearningComplete=0}
  state MoogStateMachine [parallel]
    settings: executionOrder=1
    state Initialisation
      state SwitchOffDisabled
        % StatusWord= xxxx_xxxx_x0xx_0000, 0x00, 0d
        en:
        MoogSMState=13;
        ControlWord=0; % 0x00
      state Init
        en:
        MoogSMState=11;
        ControlWord=0;
        InitComplete =0;
      state ClearFault
        en:
        MoogSMState=12;
        ControlWord=128; % 0x80
      state SwitchOnDisabled
        % StatusWord= xxxx_xxxx_x1xx_0000, 0x40, 64d
        en:
        MoogSMState=14;
        ControlWord=6; % 0x06
      state ReadyToSwitchOn
        % StatusWord=xxxx_xxxx_x01x_0001, 0x21, 33d
        en:
        MoogSMState=15;
        ControlWord=7; % 0x07
      state SwitchedOn
        % StatusWord=xxxx_xxxx_x01x_0011, 0x23, 35d
        en:
        MoogSMState=16;
        ControlWord=15; % 0x0F
      state OperationEnabled
        % StatusWord=xxxx_xxxx_x01x_0111, 0x27, 39d
        en:
        MoogSMState=17;
        ControlWord=15; % 0x0F
        InitComplete=1;
      SwitchOffDisabled -> Init [order 2] : after(1,sec)[bitand(StatusWord,8)]{FaultCntr=FaultCntr+1;}
      (default) -> Init
      Init -> ClearFault : after(0.5,sec)
      ClearFault -> SwitchOffDisabled : after(0.5,sec)
      SwitchOffDisabled -> SwitchOnDisabled [order 1] : after(0.1,sec)[bitand(StatusWord,64)]
      OperationEnabled -> Init : after(1,sec)[bitand(StatusWord,8)]{FaultCntr=FaultCntr+1;}
      SwitchedOn -> Init [order 2] : after(1,sec)[bitand(StatusWord,8)]{FaultCntr=FaultCntr+1;}
      ReadyToSwitchOn -> Init [order 2] : after(1,sec)[bitand(StatusWord,8)]{FaultCntr=FaultCntr+1;}
      SwitchOnDisabled -> Init [order 2] : after(1,sec)[bitand(StatusWord,8)]{FaultCntr=FaultCntr+1;}
      SwitchOnDisabled -> ReadyToSwitchOn [order 1] : after(0.1,sec)[bitand(StatusWord,32) &...
          |  bitand(StatusWord,1)]
      ReadyToSwitchOn -> SwitchedOn [order 1] : after(0.1,sec)[bitand(StatusWord,32) & ...
          | bitand(StatusWord,2) & ...
          | bitand(StatusWord,1)]
      SwitchedOn -> OperationEnabled [order 1] : after(0.1,sec)[bitand(StatusWord,32) & ...
          | bitand(StatusWord,4) & ...
          | bitand(StatusWord,2) & ...
          | bitand(StatusWord,1)]
    state Wait
      en:
      MoogSMState=31;
      Actuator_Ready=0;
      InitComplete =0;
      LearningComplete=0;
    state PositionControl
      state EnableSetPoint
        en:
        MoogSMState=21;
        ControlWord=47; % 0x2F
      state BeginMotion
        en:
        MoogSMState=22;
        ControlWord=63; % 0x3F
      (default) -> EnableSetPoint
      EnableSetPoint -> BeginMotion : after(0.001,sec)[Actuator_Ready==1 || ...
          | MoogOpMode==21 || ...
          | MoogOpMode==31]
      BeginMotion -> EnableSetPoint : after(0.001,sec)
    Initialisation -> Wait [order 2] : after(2,sec)[CAN_CommsOK_Flg ==0]
    (default) -> Initialisation : {FaultCntr=0;}
    Initialisation -> Wait [order 3] : [FaultCntr>=5]
    Wait -> Initialisation : [ResetCmd &&CAN_CommsOK_Flg==1 ]{Actuator_Ready=0;FaultCntr=0;}
    Initialisation -> PositionControl [order 1] : [InitComplete==1]
    PositionControl -> Initialisation [order 1] : [ResetCmd ]{InitComplete=0;}
    PositionControl -> Initialisation [order 2] : [bitand(StatusWord,8)]{InitComplete=0;FaultCntr=FaultCntr+1;}
  data: CAN_CommsOK_Flg input; ControlWord output; PositionCmd output; ResetCmd input; PositionLearningTrigger input; StatusWord input; Actuator_Ready output; FaultCntr output; MoogSMState output; InitComplete output; MoogOpMode output; LearningComplete output; ActualPosition_cnt input; MaxStop output; MinStop output; TargetPosition_cnt input; ActuatorMinTravelForReady input

== matlab function EV6_LUT_FourWheel_EV6Battery77p4kWh_PowerCorrected/Vehicle Under Test1/Vehicle/Rototest and ORNL Interface/Get Wheel Spd Cmd Based on Wheel Dynamics/Whl Dynamics & Format CM Powertrain Signal/Subsystem/MATLAB Function ==
  data: axleTorq input; switchFlag output; wheelSpd input
function switchFlag = fcn(axleTorq, wheelSpd)

% if braking and vehicle has stopped
if (abs(axleTorq) < 1e-5 && abs(wheelSpd) < 1e-5)
    switchFlag = 1;
else
    switchFlag = 0;
end

== matlab function EV6_LUT_FourWheel_EV6Battery77p4kWh_PowerCorrected/Vehicle Under Test1/Vehicle/Rototest and ORNL Interface/Get Wheel Spd Cmd Based on Wheel Dynamics/Whl Dynamics & Format CM Powertrain Signal/Subsystem2/MATLAB Function ==
  data: axleTorq input; switchFlag output; wheelSpd input
function switchFlag = fcn(axleTorq, wheelSpd)

% if braking and vehicle has stopped
if (abs(axleTorq) < 1e-5 && abs(wheelSpd) < 1e-5)
    switchFlag = 1;
else
    switchFlag = 0;
end

== matlab function EV6_LUT_FourWheel_EV6Battery77p4kWh_PowerCorrected/Vehicle Under Test1/Vehicle/Rototest and ORNL Interface/Get Wheel Spd Cmd Based on Wheel Dynamics/Whl Dynamics & Format CM Powertrain Signal/Subsystem3/MATLAB Function ==
  data: axleTorq input; switchFlag output; wheelSpd input
function switchFlag = fcn(axleTorq, wheelSpd)

% if braking and vehicle has stopped
if (abs(axleTorq) < 1e-5 && abs(wheelSpd) < 1e-5)
    switchFlag = 1;
else
    switchFlag = 0;
end

== matlab function EV6_LUT_FourWheel_EV6Battery77p4kWh_PowerCorrected/Vehicle Under Test1/Vehicle/Rototest and ORNL Interface/Get Wheel Spd Cmd Based on Wheel Dynamics/Whl Dynamics & Format CM Powertrain Signal/Subsystem4/MATLAB Function ==
  data: axleTorq input; switchFlag output; wheelSpd input
function switchFlag = fcn(axleTorq, wheelSpd)

% if braking and vehicle has stopped
if (abs(axleTorq) < 1e-5 && abs(wheelSpd) < 1e-5)
    switchFlag = 1;
else
    switchFlag = 0;
end
